simulink model "simulink_scheme_task_41"  (R2023b)
settings: Solver=VariableStepAuto  StartTime=0.0  StopTime=10.0  RelTol=1e-3
values from neighbouring files (symbols this model uses):
  nInput = size(B,2)    [buildCondMatrices.m]    (also in main_task41.m; main_task42.m)
  patientParameters = loadPatientParameter(sprintf('patient#    [main_task41.m]    (also in main_task42.m)
  predictedHorizon = 100    [main_task41.m]    (also in main_task42.m)
  predictionData = buildCondMatrices(A_aug,B_aug,C_aug,Q,R,predictedHorizon)    [main_task41.m]    (also in main_task42.m)
  simulationParameters = loadSimulationParameter    [main_task41.m]    (also in main_task42.m)
undefined symbols (not defined in the file or in its folder): MPCctrl_fvf
settings Model: Creator=william  LastModifiedBy=william
settings DataIOCC: ReturnWorkspaceOutputs=off
settings RTWCC: GPUComputeCapability=5.0
settings ConfigComp: CovBoundaryAbsTol=1.0e-5

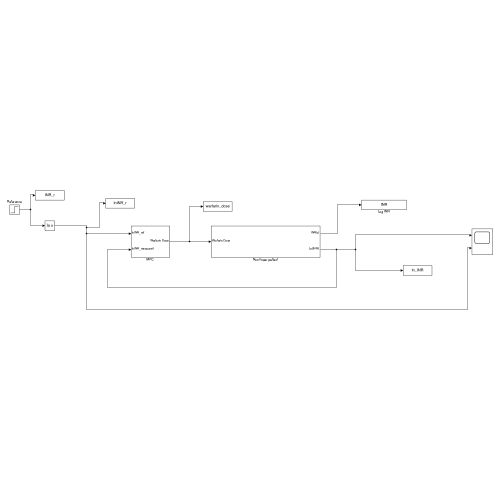
[thumbnail: Simulink's stored preview of the top-level diagram]
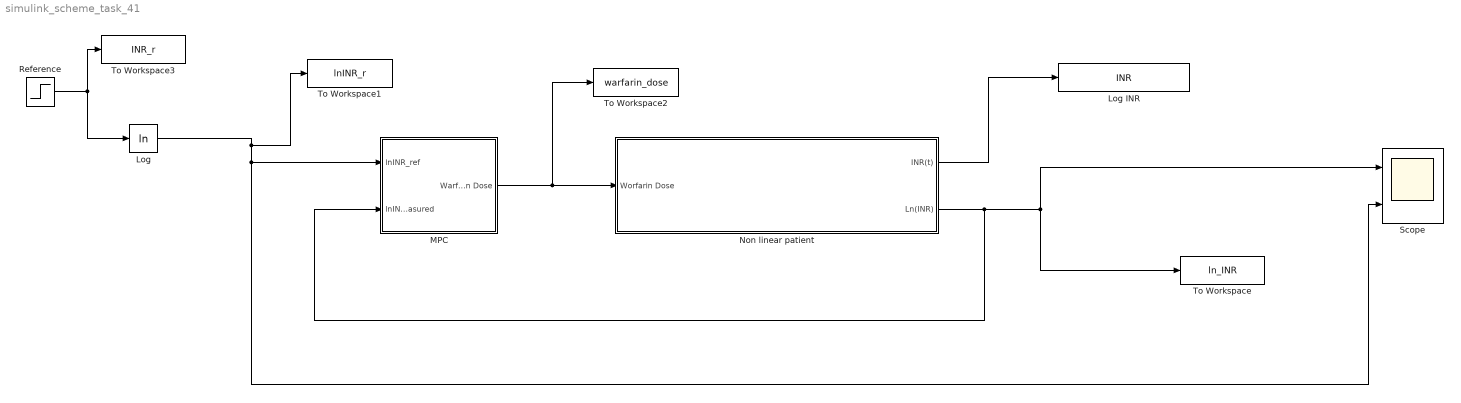
== system simulink_scheme_task_41 ==
  Log : Math  Operator=log
  Log INR : ToWorkspace  VariableName=INR  SaveFormat=Structure With Time  SampleTime=-1
  MPC : Subsystem
  Non linear patient : Subsystem
  Reference : Step  Time=2*24  Before=1  After=2.5  SampleTime=simulationParameters.Ts
  Scope : Scope  NumInputPorts=2
  To Workspace : ToWorkspace  VariableName=ln_INR  SaveFormat=Structure With Time  SampleTime=-1
  To Workspace1 : ToWorkspace  VariableName=lnINR_r  SaveFormat=Structure With Time  SampleTime=-1
  To Workspace2 : ToWorkspace  VariableName=warfarin_dose  SaveFormat=Structure With Time  SampleTime=-1
  To Workspace3 : ToWorkspace  VariableName=INR_r  SaveFormat=Structure With Time  SampleTime=-1
  wires:
  Reference/1 -> Log/1, To Workspace3/1
  Log/1 -> To Workspace1/1, MPC/1(lnINR_ref), Scope/2
  MPC/1(Warfarin Dose) -> To Workspace2/1, Non linear patient/1(Worfarin Dose)
  Non linear patient/2(Ln(INR)) -> MPC/2(lnINR_measured), Scope/1, To Workspace/1
  Non linear patient/1(INR(t)) -> Log INR/1

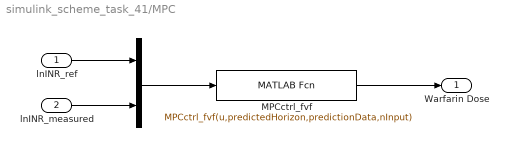
== system simulink_scheme_task_41/MPC ==
  lnINR_ref : Inport
  lnINR_measured : Inport  Port=2
  " " : Mux  Inputs=2
  MPCctrl_fvf : MATLABFcn  MATLABFcn=MPCctrl_fvf(u,predictedHorizon,predictionData,nInput)  OutputDimensions=nInput
  Warfarin Dose : Outport
  wires:
  " "/1 -> MPCctrl_fvf/1
  lnINR_measured/1 -> " "/2
  MPCctrl_fvf/1 -> Warfarin Dose/1
  lnINR_ref/1 -> " "/1

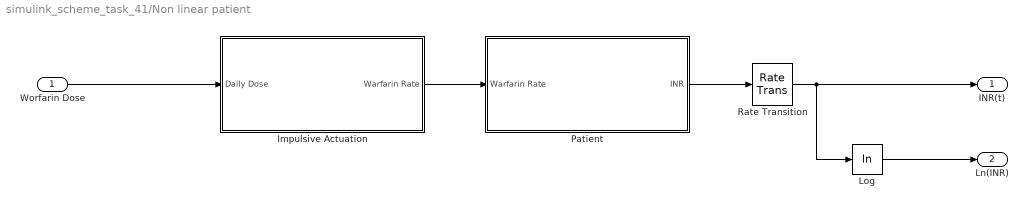
== system simulink_scheme_task_41/Non linear patient ==
  Worfarin Dose : Inport
  Impulsive Actuation : Subsystem
  Log : Math  Operator=log
  Patient : Subsystem
  Rate Transition : RateTransition  InitialCondition=patientParameters.BASE  OutPortSampleTime=simulationParameters.Ts
  INR(t) : Outport
  Ln(INR) : Outport  Port=2
  wires:
  Rate Transition/1 -> INR(t)/1, Log/1
  Log/1 -> Ln(INR)/1
  Patient/1(INR) -> Rate Transition/1
  Impulsive Actuation/1(Warfarin Rate) -> Patient/1(Warfarin Rate)
  Worfarin Dose/1 -> Impulsive Actuation/1(Daily Dose)

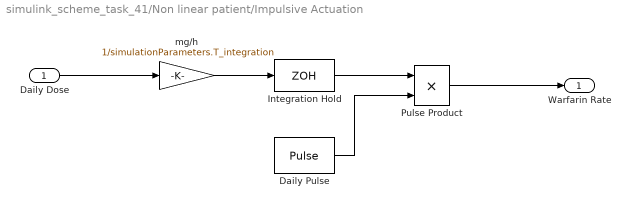
== system simulink_scheme_task_41/Non linear patient/Impulsive Actuation ==
  Daily Dose : Inport
  Daily Pulse : DiscretePulseGenerator  Period=simulationParameters.Ts/simulationParameters.T_integration  SampleTime=simulationParameters.T_integration
  Integration Hold : ZeroOrderHold  SampleTime=simulationParameters.T_integration
  Pulse Product : Product  Inputs=**
  mg/h : Gain  Gain=1/simulationParameters.T_integration
  Warfarin Rate : Outport
  wires:
  Pulse Product/1 -> Warfarin Rate/1
  Integration Hold/1 -> Pulse Product/1
  mg/h/1 -> Integration Hold/1
  Daily Dose/1 -> mg/h/1
  Daily Pulse/1 -> Pulse Product/2

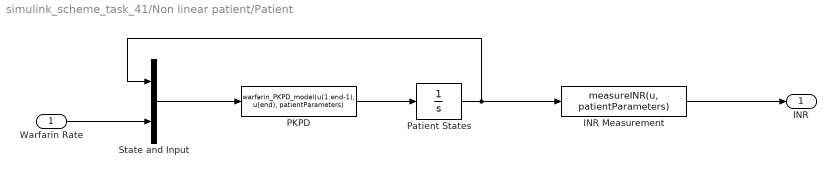
== system simulink_scheme_task_41/Non linear patient/Patient ==
  Warfarin Rate : Inport
  INR Measurement : MATLABFcn  MATLABFcn=measureINR(u, patientParameters)
  PKPD : MATLABFcn  MATLABFcn=warfarin_PKPD_model(u(1:end-1), u(end), patientParameters)  OutputDimensions=8
  Patient States : Integrator  InitialCondition=[patientParameters.x0,patientParameters.appearance.x0]
  State and Input : Mux  Inputs=2
  INR : Outport
  wires:
  Patient States/1 -> State and Input/1, INR Measurement/1
  Warfarin Rate/1 -> State and Input/2
  PKPD/1 -> Patient States/1
  INR Measurement/1 -> INR/1
  State and Input/1 -> PKPD/1
